simulink model "sys1"  (R2023b)
settings: Solver=VariableStepAuto  StartTime=0.0  StopTime=30e-3  RelTol=1e-3
InitFcn:
  | fs = 100e6;
  | ts = 1 / fs;
values from neighbouring files (symbols this model uses):
  c = 3e8    (= 300000000)    [init_param.m]
  H_az1 = zeros(numSamples,numPulses)    [init_param.m]
  H_az2 = zeros(numSamples,numPulses)    [init_param.m]
  H_ref = fft(conj(fliplr(txChirp)), numSamples)    [init_param.m]
  rawData = rawData + 0.01 * (randn(size(rawData)) + 1j * randn(size(rawData)))    [init_param.m]
  x1 = zeros(size(rawData))    [main.m]
  x2 = zeros(size(x1))    [main.m]
  x3 = zeros(size(x2))    [main.m]
  x4 = zeros(size(x3))    [main.m]
  x5 = zeros(size(x4))    [main.m]
  x6 = zeros(size(x5))    [main.m]
  xx4 = zeros(size(xx3))    [main.m]
  xx5 = zeros(size(xx4))    [main.m]
  xx6 = zeros(size(xx5))    [main.m]
undefined symbols (not defined in the file or in its folder): ffva1156, w2, w3, w4, w5, w6, w7, w8, w9, ww2, ww3, ww4, ww5, ww6, ww7, ww8, ww9, xcku095
libraries: hdlBasic x917, hdlDSPIP x18, dspsrcs4 x12, vmcUtilities x1
(part 6 of 9)

== system sys1/SAR/stream/stream_fft/stage8/BF ==
  re2 : Inport
  im2 : Inport  Port=2
  re1 : Inport  Port=3
  im1 : Inport  Port=4
  AddSub1 : hdlBasic/AddSub  mode=Addition  use_carryin=off  use_carryout=off  en=off  latency=0  precision=User Defined  arith_type="Signed  (2's comp)"  n_bits=16  bin_pt=0  quantization="Round  (unbiased: +/- Inf)"  overflow=Flag as error  use_behavioral_HDL=off  hw_selection=Fabric  pipelined=off  XmcBlockStatus=1  maskContainerNames=tabcontainer1  block_type=addsub  block_config=sysgen:Addsub_config
  AddSub2 : hdlBasic/AddSub  mode=Addition  use_carryin=off  use_carryout=off  en=off  latency=0  precision=User Defined  arith_type="Signed  (2's comp)"  n_bits=16  bin_pt=0  quantization="Round  (unbiased: +/- Inf)"  overflow=Flag as error  use_behavioral_HDL=off  hw_selection=Fabric  pipelined=off  XmcBlockStatus=1  maskContainerNames=tabcontainer1  block_type=addsub  block_config=sysgen:Addsub_config
  AddSub3 : hdlBasic/AddSub  mode=Subtraction  use_carryin=off  use_carryout=off  en=off  latency=0  precision=User Defined  arith_type="Signed  (2's comp)"  n_bits=16  bin_pt=0  quantization="Round  (unbiased: +/- Inf)"  overflow=Flag as error  use_behavioral_HDL=off  hw_selection=Fabric  pipelined=off  XmcBlockStatus=1  maskContainerNames=tabcontainer1  block_type=addsub  block_config=sysgen:Addsub_config
  AddSub4 : hdlBasic/AddSub  mode=Subtraction  use_carryin=off  use_carryout=off  en=off  latency=0  precision=User Defined  arith_type="Signed  (2's comp)"  n_bits=16  bin_pt=0  quantization="Round  (unbiased: +/- Inf)"  overflow=Flag as error  use_behavioral_HDL=off  hw_selection=Fabric  pipelined=off  XmcBlockStatus=1  maskContainerNames=tabcontainer1  block_type=addsub  block_config=sysgen:Addsub_config
  Delay2 : hdlBasic/Delay  rst=off  en=off  latency=7  reg_retiming=off  XmcBlockStatus=1  maskContainerNames=group1  block_type=delay  block_config=sysgen:Delay_config
  Delay3 : hdlBasic/Delay  rst=off  en=off  latency=7  reg_retiming=off  XmcBlockStatus=1  maskContainerNames=group1  block_type=delay  block_config=sysgen:Delay_config
  Out2_r : Outport
  Out2_i : Outport  Port=2
  Out1_r : Outport  Port=3
  Out1_i : Outport  Port=4
  wires:
  Delay3/1 -> Out2_i/1
  Delay2/1 -> Out2_r/1
  im1/1 -> AddSub3/2, AddSub1/2
  re1/1 -> AddSub4/2, AddSub2/2
  AddSub1/1 -> Delay3/1
  AddSub2/1 -> Delay2/1
  im2/1 -> AddSub3/1, AddSub1/1
  re2/1 -> AddSub4/1, AddSub2/1
  AddSub3/1 -> Out1_i/1
  AddSub4/1 -> Out1_r/1

== system sys1/SAR/stream/stream_fft/stage8/Multiplexer ==
  r1 : Inport
  i1 : Inport  Port=2
  r2 : Inport  Port=3
  i2 : Inport  Port=4
  cnt : Inport  Port=5
  BitBasher : hdlBasic/BitBasher  bitexpr=a={b[17]}  display_expr=off  sr_1=a  arith_type1=Unsigned  bin_pt1=0  sr_2=2  arith_type2=Unsigned  bin_pt2=0  sr_3=3  arith_type3=Unsigned  bin_pt3=0  sr_4=4  arith_type4=Unsigned  bin_pt4=0  XmcBlockStatus=1  maskContainerNames=group1  block_type=bitbasher  block_config=sysgen:BitBasher_config
  Inverter : hdlBasic/Inverter  en=off  latency=0  XmcBlockStatus=1  maskContainerNames=group2  block_type=inv  block_config=sysgen:Inverter_config
  Mux : hdlBasic/Mux  inputs=2  en=off  latency=0  precision=Full  arith_type=Unsigned  n_bits=16  bin_pt=14  quantization=Truncate  overflow=Wrap  XmcBlockStatus=1  maskContainerNames=tabcontainer1  block_type=mux  block_config=sysgen:Mux_config
  Mux1 : hdlBasic/Mux  inputs=2  en=off  latency=0  precision=Full  arith_type=Unsigned  n_bits=16  bin_pt=14  quantization=Truncate  overflow=Wrap  XmcBlockStatus=1  maskContainerNames=tabcontainer1  block_type=mux  block_config=sysgen:Mux_config
  rr : Outport
  ii : Outport  Port=2
  wires:
  Inverter/1 -> Mux1/1, Mux/1
  cnt/1 -> BitBasher/1
  Mux/1 -> rr/1
  Mux1/1 -> ii/1
  i1/1 -> Mux1/3
  r2/1 -> Mux/2
  BitBasher/1 -> Inverter/1
  i2/1 -> Mux1/2
  r1/1 -> Mux/3

== system sys1/SAR/stream/stream_fft/stage8/Twiddle ==
  r : Inport
  i : Inport  Port=2
  cnt : Inport  Port=3
  BitBasher1 : hdlBasic/BitBasher  bitexpr=a={b[16:10]}  display_expr=off  sr_1=a  arith_type1=Unsigned  bin_pt1=0  sr_2=2  arith_type2=Unsigned  bin_pt2=0  sr_3=3  arith_type3=Unsigned  bin_pt3=0  sr_4=4  arith_type4=Unsigned  bin_pt4=0  XmcBlockStatus=1  maskContainerNames=group1  block_type=bitbasher  block_config=sysgen:BitBasher_config
  Complex Multiplier 6.0 : hdlDSPIP/Complex Multiplier 6.0   hasatlast=off  hasatuser=off  atuserwidth=1  hasbtlast=off  hasbtuser=off  btuserwidth=1  multtype=Use_Mults  optimizegoal=Resources  flowcontrol=NonBlocking  outputwidth=32  roundmode=Truncate  hasctrltlast=off  hasctrltuser=off  ctrltuserwidth=1  outtlastbehv=Null  latencyconfig=Manual  minimumlatency=6  aclken=off  aresetn=off  trim_axipin_name=on  simulation_type=hybrid_sim  simulation_model=sysgen:cmpy_v6_0  data_path_portlist={ 's_axis_a_tdata_real', 's_axis_a_tdata_imag', 's_axis_b_tdata_real', 's_axis_b_tdata_imag', 's_axis_ctrl_tdata_rounding_bit', 'm_axis_dout_tdata_real', 'm_axis_dout_tdata_imag' }  aportwidth=63  bportwidth=63  ip_name=Complex Multiplier  ip_version=6.0  dsptool_ready=true  ipcore_usecache=true  ipcore_useipmodelcache=true  ipcore_verbose=false  ipcore_latency_parameter='minimumlatency'  wrapper_available=true  port_translation_map={ 'aclken' => 'en', 'aresetn' => 'rst'}  XmcBlockStatus=1  maskContainerNames=tabcontainer1  block_type=cmpy_v6_0  block_config=sysgen:rodinimport_config
  Constant2 : hdlBasic/Constant  const=1  gui_display_data_type=Boolean  arith_type=Boolean  n_bits=16  bin_pt=14  preci_type=Single  exp_width=8  frac_width=24  explicit_period=on  period=ts  XmcBlockStatus=1  maskContainerNames=tabcontainer1  block_type=constant  block_config=sysgen:Constant_config
  Constant3 : hdlBasic/Constant  const=1  gui_display_data_type=Boolean  arith_type=Boolean  n_bits=16  bin_pt=14  preci_type=Single  exp_width=8  frac_width=24  explicit_period=on  period=ts  XmcBlockStatus=1  maskContainerNames=tabcontainer1  block_type=constant  block_config=sysgen:Constant_config
  Convert1 : hdlBasic/Convert  gui_display_data_type=Fixed-point  arith_type=Signed (2's comp)  n_bits=16  bin_pt=0  float_type=Single  exp_bits=8  fraction_bits=24  quantization=Truncate  overflow=Flag as error  en=off  latency=0  pipeline=off  XmcBlockStatus=1  maskContainerNames=group2  block_type=convert  block_config=sysgen:Convert_config  block_width=595  block_height=885
  Convert2 : hdlBasic/Convert  gui_display_data_type=Fixed-point  arith_type=Signed (2's comp)  n_bits=16  bin_pt=0  float_type=Single  exp_bits=8  fraction_bits=24  quantization=Truncate  overflow=Flag as error  en=off  latency=0  pipeline=off  XmcBlockStatus=1  maskContainerNames=group2  block_type=convert  block_config=sysgen:Convert_config  block_width=595  block_height=885
  Delay2 : hdlBasic/Delay  rst=off  en=off  latency=1  reg_retiming=off  XmcBlockStatus=1  maskContainerNames=group1  block_type=delay  block_config=sysgen:Delay_config
  Delay3 : hdlBasic/Delay  rst=off  en=off  latency=1  reg_retiming=off  XmcBlockStatus=1  maskContainerNames=group1  block_type=delay  block_config=sysgen:Delay_config
  ROM : hdlBasic/ROM  depth=length(w8)  initVector=real(w8)  distributed_mem=Block RAM  rst=off  init_reg=0  en=off  latency=1  gui_display_data_type=Fixed-point  arith_type="Signed  (2's comp)"  n_bits=16  bin_pt=15  preci_type=Single  exp_width=8  frac_width=24  optimize=Area  use_rpm=on  simulation_type=fast_sim  XmcBlockStatus=1  maskContainerNames=tabcontainer1  block_type=sprom  block_config=sysgen:SPROM_config
  ROM1 : hdlBasic/ROM  depth=length(w8)  initVector=imag(w8)  distributed_mem=Block RAM  rst=off  init_reg=0  en=off  latency=1  gui_display_data_type=Fixed-point  arith_type="Signed  (2's comp)"  n_bits=16  bin_pt=15  preci_type=Single  exp_width=8  frac_width=24  optimize=Area  use_rpm=on  simulation_type=fast_sim  XmcBlockStatus=1  maskContainerNames=tabcontainer1  block_type=sprom  block_config=sysgen:SPROM_config
  rr : Outport
  ii : Outport  Port=2
  wires:
  Delay3/1 -> Complex Multiplier 6.0/3
  Delay2/1 -> Complex Multiplier 6.0/2
  Convert1/1 -> rr/1
  Convert2/1 -> ii/1
  cnt/1 -> BitBasher1/1
  r/1 -> Delay3/1
  Complex Multiplier 6.0/3 -> Convert1/1
  i/1 -> Delay2/1
  Constant3/1 -> Complex Multiplier 6.0/4
  ROM/1 -> Complex Multiplier 6.0/6
  Constant2/1 -> Complex Multiplier 6.0/1
  Complex Multiplier 6.0/2 -> Convert2/1
  BitBasher1/1 -> ROM1/1, ROM/1
  ROM1/1 -> Complex Multiplier 6.0/5

== system sys1/SAR/stream/stream_fft/stage8/delay ==
  r : Inport
  i : Inport  Port=2
  cnt : Inport  Port=3
  r1 : Inport  Port=4
  i1 : Inport  Port=5
  BitBasher : hdlBasic/BitBasher  bitexpr=a={b[17]}  display_expr=off  sr_1=a  arith_type1=Unsigned  bin_pt1=0  sr_2=2  arith_type2=Unsigned  bin_pt2=0  sr_3=3  arith_type3=Unsigned  bin_pt3=0  sr_4=4  arith_type4=Unsigned  bin_pt4=0  XmcBlockStatus=1  maskContainerNames=group1  block_type=bitbasher  block_config=sysgen:BitBasher_config
  Inverter : hdlBasic/Inverter  en=off  latency=0  XmcBlockStatus=1  maskContainerNames=group2  block_type=inv  block_config=sysgen:Inverter_config
  Mux : hdlBasic/Mux  inputs=2  en=off  latency=0  precision=Full  arith_type=Unsigned  n_bits=16  bin_pt=14  quantization=Truncate  overflow=Wrap  XmcBlockStatus=1  maskContainerNames=tabcontainer1  block_type=mux  block_config=sysgen:Mux_config
  Mux1 : hdlBasic/Mux  inputs=2  en=off  latency=0  precision=Full  arith_type=Unsigned  n_bits=16  bin_pt=14  quantization=Truncate  overflow=Wrap  XmcBlockStatus=1  maskContainerNames=tabcontainer1  block_type=mux  block_config=sysgen:Mux_config
  delay : Subsystem
  delay1 : Subsystem
  rr : Outport
  ii : Outport  Port=2
  wires:
  i/1 -> Mux1/3
  r/1 -> Mux/3
  delay1/1(out) -> ii/1
  delay/1(out) -> rr/1
  i1/1 -> Mux1/2
  r1/1 -> Mux/2
  Mux1/1 -> delay1/1(in)
  Mux/1 -> delay/1(in)
  BitBasher/1 -> Inverter/1
  cnt/1 -> BitBasher/1
  Inverter/1 -> Mux/1, Mux1/1

== system sys1/SAR/stream/stream_fft/stage9/BF ==
  re2 : Inport
  im2 : Inport  Port=2
  re1 : Inport  Port=3
  im1 : Inport  Port=4
  AddSub1 : hdlBasic/AddSub  mode=Addition  use_carryin=off  use_carryout=off  en=off  latency=0  precision=User Defined  arith_type="Signed  (2's comp)"  n_bits=16  bin_pt=0  quantization="Round  (unbiased: +/- Inf)"  overflow=Flag as error  use_behavioral_HDL=off  hw_selection=Fabric  pipelined=off  XmcBlockStatus=1  maskContainerNames=tabcontainer1  block_type=addsub  block_config=sysgen:Addsub_config
  AddSub2 : hdlBasic/AddSub  mode=Addition  use_carryin=off  use_carryout=off  en=off  latency=0  precision=User Defined  arith_type="Signed  (2's comp)"  n_bits=16  bin_pt=0  quantization="Round  (unbiased: +/- Inf)"  overflow=Flag as error  use_behavioral_HDL=off  hw_selection=Fabric  pipelined=off  XmcBlockStatus=1  maskContainerNames=tabcontainer1  block_type=addsub  block_config=sysgen:Addsub_config
  AddSub3 : hdlBasic/AddSub  mode=Subtraction  use_carryin=off  use_carryout=off  en=off  latency=0  precision=User Defined  arith_type="Signed  (2's comp)"  n_bits=16  bin_pt=0  quantization="Round  (unbiased: +/- Inf)"  overflow=Flag as error  use_behavioral_HDL=off  hw_selection=Fabric  pipelined=off  XmcBlockStatus=1  maskContainerNames=tabcontainer1  block_type=addsub  block_config=sysgen:Addsub_config
  AddSub4 : hdlBasic/AddSub  mode=Subtraction  use_carryin=off  use_carryout=off  en=off  latency=0  precision=User Defined  arith_type="Signed  (2's comp)"  n_bits=16  bin_pt=0  quantization="Round  (unbiased: +/- Inf)"  overflow=Flag as error  use_behavioral_HDL=off  hw_selection=Fabric  pipelined=off  XmcBlockStatus=1  maskContainerNames=tabcontainer1  block_type=addsub  block_config=sysgen:Addsub_config
  Delay2 : hdlBasic/Delay  rst=off  en=off  latency=7  reg_retiming=off  XmcBlockStatus=1  maskContainerNames=group1  block_type=delay  block_config=sysgen:Delay_config
  Delay3 : hdlBasic/Delay  rst=off  en=off  latency=7  reg_retiming=off  XmcBlockStatus=1  maskContainerNames=group1  block_type=delay  block_config=sysgen:Delay_config
  Out2_r : Outport
  Out2_i : Outport  Port=2
  Out1_r : Outport  Port=3
  Out1_i : Outport  Port=4
  wires:
  AddSub4/1 -> Out1_r/1
  AddSub3/1 -> Out1_i/1
  re2/1 -> AddSub2/1, AddSub4/1
  im2/1 -> AddSub1/1, AddSub3/1
  AddSub2/1 -> Delay2/1
  AddSub1/1 -> Delay3/1
  re1/1 -> AddSub2/2, AddSub4/2
  im1/1 -> AddSub1/2, AddSub3/2
  Delay2/1 -> Out2_r/1
  Delay3/1 -> Out2_i/1

== system sys1/SAR/stream/stream_fft/stage9/Multiplexer ==
  r1 : Inport
  i1 : Inport  Port=2
  r2 : Inport  Port=3
  i2 : Inport  Port=4
  cnt : Inport  Port=5
  BitBasher : hdlBasic/BitBasher  bitexpr=a={b[18]}  display_expr=off  sr_1=a  arith_type1=Unsigned  bin_pt1=0  sr_2=2  arith_type2=Unsigned  bin_pt2=0  sr_3=3  arith_type3=Unsigned  bin_pt3=0  sr_4=4  arith_type4=Unsigned  bin_pt4=0  XmcBlockStatus=1  maskContainerNames=group1  block_type=bitbasher  block_config=sysgen:BitBasher_config
  Inverter : hdlBasic/Inverter  en=off  latency=0  XmcBlockStatus=1  maskContainerNames=group2  block_type=inv  block_config=sysgen:Inverter_config
  Mux : hdlBasic/Mux  inputs=2  en=off  latency=0  precision=Full  arith_type=Unsigned  n_bits=16  bin_pt=14  quantization=Truncate  overflow=Wrap  XmcBlockStatus=1  maskContainerNames=tabcontainer1  block_type=mux  block_config=sysgen:Mux_config
  Mux1 : hdlBasic/Mux  inputs=2  en=off  latency=0  precision=Full  arith_type=Unsigned  n_bits=16  bin_pt=14  quantization=Truncate  overflow=Wrap  XmcBlockStatus=1  maskContainerNames=tabcontainer1  block_type=mux  block_config=sysgen:Mux_config
  rr : Outport
  ii : Outport  Port=2
  wires:
  r1/1 -> Mux/3
  i2/1 -> Mux1/2
  BitBasher/1 -> Inverter/1
  r2/1 -> Mux/2
  i1/1 -> Mux1/3
  Mux1/1 -> ii/1
  Mux/1 -> rr/1
  cnt/1 -> BitBasher/1
  Inverter/1 -> Mux/1, Mux1/1

== system sys1/SAR/stream/stream_fft/stage9/Twiddle ==
  r : Inport
  i : Inport  Port=2
  cnt : Inport  Port=3
  BitBasher1 : hdlBasic/BitBasher  bitexpr=a={b[17:10]}  display_expr=off  sr_1=a  arith_type1=Unsigned  bin_pt1=0  sr_2=2  arith_type2=Unsigned  bin_pt2=0  sr_3=3  arith_type3=Unsigned  bin_pt3=0  sr_4=4  arith_type4=Unsigned  bin_pt4=0  XmcBlockStatus=1  maskContainerNames=group1  block_type=bitbasher  block_config=sysgen:BitBasher_config
  Complex Multiplier 6.0 : hdlDSPIP/Complex Multiplier 6.0   hasatlast=off  hasatuser=off  atuserwidth=1  hasbtlast=off  hasbtuser=off  btuserwidth=1  multtype=Use_Mults  optimizegoal=Resources  flowcontrol=NonBlocking  outputwidth=32  roundmode=Truncate  hasctrltlast=off  hasctrltuser=off  ctrltuserwidth=1  outtlastbehv=Null  latencyconfig=Manual  minimumlatency=6  aclken=off  aresetn=off  trim_axipin_name=on  simulation_type=hybrid_sim  simulation_model=sysgen:cmpy_v6_0  data_path_portlist={ 's_axis_a_tdata_real', 's_axis_a_tdata_imag', 's_axis_b_tdata_real', 's_axis_b_tdata_imag', 's_axis_ctrl_tdata_rounding_bit', 'm_axis_dout_tdata_real', 'm_axis_dout_tdata_imag' }  aportwidth=63  bportwidth=63  ip_name=Complex Multiplier  ip_version=6.0  dsptool_ready=true  ipcore_usecache=true  ipcore_useipmodelcache=true  ipcore_verbose=false  ipcore_latency_parameter='minimumlatency'  wrapper_available=true  port_translation_map={ 'aclken' => 'en', 'aresetn' => 'rst'}  XmcBlockStatus=1  maskContainerNames=tabcontainer1  block_type=cmpy_v6_0  block_config=sysgen:rodinimport_config
  Constant2 : hdlBasic/Constant  const=1  gui_display_data_type=Boolean  arith_type=Boolean  n_bits=16  bin_pt=14  preci_type=Single  exp_width=8  frac_width=24  explicit_period=on  period=ts  XmcBlockStatus=1  maskContainerNames=tabcontainer1  block_type=constant  block_config=sysgen:Constant_config
  Constant3 : hdlBasic/Constant  const=1  gui_display_data_type=Boolean  arith_type=Boolean  n_bits=16  bin_pt=14  preci_type=Single  exp_width=8  frac_width=24  explicit_period=on  period=ts  XmcBlockStatus=1  maskContainerNames=tabcontainer1  block_type=constant  block_config=sysgen:Constant_config
  Convert1 : hdlBasic/Convert  gui_display_data_type=Fixed-point  arith_type=Signed (2's comp)  n_bits=16  bin_pt=0  float_type=Single  exp_bits=8  fraction_bits=24  quantization=Truncate  overflow=Flag as error  en=off  latency=0  pipeline=off  XmcBlockStatus=1  maskContainerNames=group2  block_type=convert  block_config=sysgen:Convert_config  block_width=595  block_height=885
  Convert2 : hdlBasic/Convert  gui_display_data_type=Fixed-point  arith_type=Signed (2's comp)  n_bits=16  bin_pt=0  float_type=Single  exp_bits=8  fraction_bits=24  quantization=Truncate  overflow=Flag as error  en=off  latency=0  pipeline=off  XmcBlockStatus=1  maskContainerNames=group2  block_type=convert  block_config=sysgen:Convert_config  block_width=595  block_height=885
  Delay2 : hdlBasic/Delay  rst=off  en=off  latency=1  reg_retiming=off  XmcBlockStatus=1  maskContainerNames=group1  block_type=delay  block_config=sysgen:Delay_config
  Delay3 : hdlBasic/Delay  rst=off  en=off  latency=1  reg_retiming=off  XmcBlockStatus=1  maskContainerNames=group1  block_type=delay  block_config=sysgen:Delay_config
  ROM : hdlBasic/ROM  depth=length(w9)  initVector=real(w9)  distributed_mem=Block RAM  rst=off  init_reg=0  en=off  latency=1  gui_display_data_type=Fixed-point  arith_type="Signed  (2's comp)"  n_bits=16  bin_pt=15  preci_type=Single  exp_width=8  frac_width=24  optimize=Area  use_rpm=on  simulation_type=fast_sim  XmcBlockStatus=1  maskContainerNames=tabcontainer1  block_type=sprom  block_config=sysgen:SPROM_config
  ROM1 : hdlBasic/ROM  depth=length(w9)  initVector=imag(w9)  distributed_mem=Block RAM  rst=off  init_reg=0  en=off  latency=1  gui_display_data_type=Fixed-point  arith_type="Signed  (2's comp)"  n_bits=16  bin_pt=15  preci_type=Single  exp_width=8  frac_width=24  optimize=Area  use_rpm=on  simulation_type=fast_sim  XmcBlockStatus=1  maskContainerNames=tabcontainer1  block_type=sprom  block_config=sysgen:SPROM_config
  rr : Outport
  ii : Outport  Port=2
  wires:
  ROM1/1 -> Complex Multiplier 6.0/5
  BitBasher1/1 -> ROM/1, ROM1/1
  Complex Multiplier 6.0/2 -> Convert2/1
  Constant2/1 -> Complex Multiplier 6.0/1
  ROM/1 -> Complex Multiplier 6.0/6
  Constant3/1 -> Complex Multiplier 6.0/4
  i/1 -> Delay2/1
  Complex Multiplier 6.0/3 -> Convert1/1
  r/1 -> Delay3/1
  cnt/1 -> BitBasher1/1
  Convert2/1 -> ii/1
  Convert1/1 -> rr/1
  Delay2/1 -> Complex Multiplier 6.0/2
  Delay3/1 -> Complex Multiplier 6.0/3

== system sys1/SAR/stream/stream_fft/stage9/delay ==
  r : Inport
  i : Inport  Port=2
  cnt : Inport  Port=3
  r1 : Inport  Port=4
  i1 : Inport  Port=5
  BitBasher : hdlBasic/BitBasher  bitexpr=a={b[18]}  display_expr=off  sr_1=a  arith_type1=Unsigned  bin_pt1=0  sr_2=2  arith_type2=Unsigned  bin_pt2=0  sr_3=3  arith_type3=Unsigned  bin_pt3=0  sr_4=4  arith_type4=Unsigned  bin_pt4=0  XmcBlockStatus=1  maskContainerNames=group1  block_type=bitbasher  block_config=sysgen:BitBasher_config
  Inverter : hdlBasic/Inverter  en=off  latency=0  XmcBlockStatus=1  maskContainerNames=group2  block_type=inv  block_config=sysgen:Inverter_config
  Mux : hdlBasic/Mux  inputs=2  en=off  latency=0  precision=Full  arith_type=Unsigned  n_bits=16  bin_pt=14  quantization=Truncate  overflow=Wrap  XmcBlockStatus=1  maskContainerNames=tabcontainer1  block_type=mux  block_config=sysgen:Mux_config
  Mux1 : hdlBasic/Mux  inputs=2  en=off  latency=0  precision=Full  arith_type=Unsigned  n_bits=16  bin_pt=14  quantization=Truncate  overflow=Wrap  XmcBlockStatus=1  maskContainerNames=tabcontainer1  block_type=mux  block_config=sysgen:Mux_config
  delay : Subsystem
  delay1 : Subsystem
  rr : Outport
  ii : Outport  Port=2
  wires:
  Inverter/1 -> Mux1/1, Mux/1
  cnt/1 -> BitBasher/1
  BitBasher/1 -> Inverter/1
  Mux/1 -> delay/1(in)
  Mux1/1 -> delay1/1(in)
  r1/1 -> Mux/2
  i1/1 -> Mux1/2
  delay/1(out) -> rr/1
  delay1/1(out) -> ii/1
  r/1 -> Mux/3
  i/1 -> Mux1/3

== system sys1/SAR/stream/stream_ifft/stage1/BF ==
  ur : Inport
  ui : Inport  Port=2
  vr : Inport  Port=3
  vi : Inport  Port=4
  AddSub1 : hdlBasic/AddSub  mode=Addition  use_carryin=off  use_carryout=off  en=off  latency=0  precision=User Defined  arith_type="Signed  (2's comp)"  n_bits=16  bin_pt=0  quantization="Round  (unbiased: +/- Inf)"  overflow=Flag as error  use_behavioral_HDL=off  hw_selection=Fabric  pipelined=off  XmcBlockStatus=1  maskContainerNames=tabcontainer1  block_type=addsub  block_config=sysgen:Addsub_config
  AddSub2 : hdlBasic/AddSub  mode=Addition  use_carryin=off  use_carryout=off  en=off  latency=0  precision=User Defined  arith_type="Signed  (2's comp)"  n_bits=16  bin_pt=0  quantization="Round  (unbiased: +/- Inf)"  overflow=Flag as error  use_behavioral_HDL=off  hw_selection=Fabric  pipelined=off  XmcBlockStatus=1  maskContainerNames=tabcontainer1  block_type=addsub  block_config=sysgen:Addsub_config
  AddSub3 : hdlBasic/AddSub  mode=Subtraction  use_carryin=off  use_carryout=off  en=off  latency=0  precision=User Defined  arith_type="Signed  (2's comp)"  n_bits=16  bin_pt=0  quantization="Round  (unbiased: +/- Inf)"  overflow=Flag as error  use_behavioral_HDL=off  hw_selection=Fabric  pipelined=off  XmcBlockStatus=1  maskContainerNames=tabcontainer1  block_type=addsub  block_config=sysgen:Addsub_config
  AddSub4 : hdlBasic/AddSub  mode=Subtraction  use_carryin=off  use_carryout=off  en=off  latency=0  precision=User Defined  arith_type="Signed  (2's comp)"  n_bits=16  bin_pt=0  quantization="Round  (unbiased: +/- Inf)"  overflow=Flag as error  use_behavioral_HDL=off  hw_selection=Fabric  pipelined=off  XmcBlockStatus=1  maskContainerNames=tabcontainer1  block_type=addsub  block_config=sysgen:Addsub_config
  Out2_r : Outport
  Out2_i : Outport  Port=2
  Out1_r : Outport  Port=3
  Out1_i : Outport  Port=4
  wires:
  AddSub2/1 -> Out2_r/1
  AddSub1/1 -> Out2_i/1
  AddSub3/1 -> Out1_r/1
  AddSub4/1 -> Out1_i/1
  ur/1 -> AddSub2/1, AddSub3/1
  ui/1 -> AddSub1/1, AddSub4/1
  vr/1 -> AddSub2/2, AddSub3/2
  vi/1 -> AddSub1/2, AddSub4/2

== system sys1/SAR/stream/stream_ifft/stage1/Multiplexer ==
  r2 : Inport
  i2 : Inport  Port=2
  r1 : Inport  Port=3
  i1 : Inport  Port=4
  cnt : Inport  Port=5
  BitBasher : hdlBasic/BitBasher  bitexpr=a={b[10]}  display_expr=on  sr_1=a  arith_type1=Unsigned  bin_pt1=0  sr_2=2  arith_type2=Unsigned  bin_pt2=0  sr_3=3  arith_type3=Unsigned  bin_pt3=0  sr_4=4  arith_type4=Unsigned  bin_pt4=0  XmcBlockStatus=1  maskContainerNames=group1  block_type=bitbasher  block_config=sysgen:BitBasher_config
  Delay1 : hdlBasic/Delay  rst=off  en=off  latency=7  reg_retiming=off  XmcBlockStatus=1  maskContainerNames=group1  block_type=delay  block_config=sysgen:Delay_config
  Inverter : hdlBasic/Inverter  en=off  latency=0  XmcBlockStatus=1  maskContainerNames=group2  block_type=inv  block_config=sysgen:Inverter_config
  Mux : hdlBasic/Mux  inputs=2  en=off  latency=0  precision=Full  arith_type=Unsigned  n_bits=16  bin_pt=14  quantization=Truncate  overflow=Wrap  XmcBlockStatus=1  maskContainerNames=tabcontainer1  block_type=mux  block_config=sysgen:Mux_config
  Mux1 : hdlBasic/Mux  inputs=2  en=off  latency=0  precision=Full  arith_type=Unsigned  n_bits=16  bin_pt=14  quantization=Truncate  overflow=Wrap  XmcBlockStatus=1  maskContainerNames=tabcontainer1  block_type=mux  block_config=sysgen:Mux_config
  rr : Outport
  ii : Outport  Port=2
  wires:
  Delay1/1 -> Mux1/1, Mux/1
  Inverter/1 -> Delay1/1
  r1/1 -> Mux/2
  r2/1 -> Mux/3
  i2/1 -> Mux1/3
  i1/1 -> Mux1/2
  cnt/1 -> BitBasher/1
  Mux/1 -> rr/1
  Mux1/1 -> ii/1
  BitBasher/1 -> Inverter/1

== system sys1/SAR/stream/stream_ifft/stage1/Twiddle1 ==
  r : Inport
  i : Inport  Port=2
  cnt : Inport  Port=3
  Delay1 : hdlBasic/Delay  rst=off  en=off  latency=6  reg_retiming=off  XmcBlockStatus=1  maskContainerNames=group1  block_type=delay  block_config=sysgen:Delay_config
  Delay7 : hdlBasic/Delay  rst=off  en=off  latency=6  reg_retiming=off  XmcBlockStatus=1  maskContainerNames=group1  block_type=delay  block_config=sysgen:Delay_config
  rr : Outport
  ii : Outport  Port=2
  wires:
  r/1 -> Delay1/1
  i/1 -> Delay7/1
  Delay7/1 -> ii/1
  Delay1/1 -> rr/1

== system sys1/SAR/stream/stream_ifft/stage1/delay ==
  r : Inport
  i : Inport  Port=2
  cnt : Inport  Port=3
  r1 : Inport  Port=4
  i1 : Inport  Port=5
  BitBasher : hdlBasic/BitBasher  bitexpr=a={b[10]}  display_expr=off  sr_1=a  arith_type1=Unsigned  bin_pt1=0  sr_2=2  arith_type2=Unsigned  bin_pt2=0  sr_3=3  arith_type3=Unsigned  bin_pt3=0  sr_4=4  arith_type4=Unsigned  bin_pt4=0  XmcBlockStatus=1  maskContainerNames=group1  block_type=bitbasher  block_config=sysgen:BitBasher_config
  Delay4 : hdlBasic/Delay  rst=off  en=off  latency=6  reg_retiming=off  XmcBlockStatus=1  maskContainerNames=group1  block_type=delay  block_config=sysgen:Delay_config
  Delay6 : hdlBasic/Delay  rst=off  en=off  latency=6  reg_retiming=off  XmcBlockStatus=1  maskContainerNames=group1  block_type=delay  block_config=sysgen:Delay_config
  Delay9 : hdlBasic/Delay  rst=off  en=off  latency=7  reg_retiming=off  XmcBlockStatus=1  maskContainerNames=group1  block_type=delay  block_config=sysgen:Delay_config
  Inverter : hdlBasic/Inverter  en=off  latency=0  XmcBlockStatus=1  maskContainerNames=group2  block_type=inv  block_config=sysgen:Inverter_config
  Mux : hdlBasic/Mux  inputs=2  en=off  latency=0  precision=Full  arith_type=Unsigned  n_bits=16  bin_pt=14  quantization=Truncate  overflow=Wrap  XmcBlockStatus=1  maskContainerNames=tabcontainer1  block_type=mux  block_config=sysgen:Mux_config
  Mux1 : hdlBasic/Mux  inputs=2  en=off  latency=0  precision=Full  arith_type=Unsigned  n_bits=16  bin_pt=14  quantization=Truncate  overflow=Wrap  XmcBlockStatus=1  maskContainerNames=tabcontainer1  block_type=mux  block_config=sysgen:Mux_config
  delay : Subsystem
  delay1 : Subsystem
  rr : Outport
  ii : Outport  Port=2
  wires:
  Delay6/1 -> Mux1/3
  Delay4/1 -> Mux/3
  Delay9/1 -> Mux1/1, Mux/1
  r1/1 -> Mux/2
  i/1 -> Delay6/1
  Mux1/1 -> delay1/1(in)
  BitBasher/1 -> Inverter/1
  i1/1 -> Mux1/2
  r/1 -> Delay4/1
  delay/1(out) -> rr/1
  delay1/1(out) -> ii/1
  Mux/1 -> delay/1(in)
  cnt/1 -> BitBasher/1
  Inverter/1 -> Delay9/1

== system sys1/SAR/stream/stream_ifft/stage2/BF ==
  ur : Inport
  ui : Inport  Port=2
  vr : Inport  Port=3
  vi : Inport  Port=4
  AddSub1 : hdlBasic/AddSub  mode=Addition  use_carryin=off  use_carryout=off  en=off  latency=0  precision=User Defined  arith_type="Signed  (2's comp)"  n_bits=16  bin_pt=0  quantization="Round  (unbiased: +/- Inf)"  overflow=Flag as error  use_behavioral_HDL=off  hw_selection=Fabric  pipelined=off  XmcBlockStatus=1  maskContainerNames=tabcontainer1  block_type=addsub  block_config=sysgen:Addsub_config
  AddSub2 : hdlBasic/AddSub  mode=Addition  use_carryin=off  use_carryout=off  en=off  latency=0  precision=User Defined  arith_type="Signed  (2's comp)"  n_bits=16  bin_pt=0  quantization="Round  (unbiased: +/- Inf)"  overflow=Flag as error  use_behavioral_HDL=off  hw_selection=Fabric  pipelined=off  XmcBlockStatus=1  maskContainerNames=tabcontainer1  block_type=addsub  block_config=sysgen:Addsub_config
  AddSub3 : hdlBasic/AddSub  mode=Subtraction  use_carryin=off  use_carryout=off  en=off  latency=0  precision=User Defined  arith_type="Signed  (2's comp)"  n_bits=16  bin_pt=0  quantization="Round  (unbiased: +/- Inf)"  overflow=Flag as error  use_behavioral_HDL=off  hw_selection=Fabric  pipelined=off  XmcBlockStatus=1  maskContainerNames=tabcontainer1  block_type=addsub  block_config=sysgen:Addsub_config
  AddSub4 : hdlBasic/AddSub  mode=Subtraction  use_carryin=off  use_carryout=off  en=off  latency=0  precision=User Defined  arith_type="Signed  (2's comp)"  n_bits=16  bin_pt=0  quantization="Round  (unbiased: +/- Inf)"  overflow=Flag as error  use_behavioral_HDL=off  hw_selection=Fabric  pipelined=off  XmcBlockStatus=1  maskContainerNames=tabcontainer1  block_type=addsub  block_config=sysgen:Addsub_config
  Out2_r : Outport
  Out2_i : Outport  Port=2
  Out1_r : Outport  Port=3
  Out1_i : Outport  Port=4
  wires:
  AddSub2/1 -> Out2_r/1
  AddSub1/1 -> Out2_i/1
  AddSub3/1 -> Out1_r/1
  AddSub4/1 -> Out1_i/1
  ur/1 -> AddSub2/1, AddSub3/1
  ui/1 -> AddSub1/1, AddSub4/1
  vr/1 -> AddSub2/2, AddSub3/2
  vi/1 -> AddSub1/2, AddSub4/2

== system sys1/SAR/stream/stream_ifft/stage2/Multiplexer ==
  r2 : Inport
  i2 : Inport  Port=2
  r1 : Inport  Port=3
  i1 : Inport  Port=4
  cnt : Inport  Port=5
  BitBasher : hdlBasic/BitBasher  bitexpr=a={b[11]}  display_expr=on  sr_1=a  arith_type1=Unsigned  bin_pt1=0  sr_2=2  arith_type2=Unsigned  bin_pt2=0  sr_3=3  arith_type3=Unsigned  bin_pt3=0  sr_4=4  arith_type4=Unsigned  bin_pt4=0  XmcBlockStatus=1  maskContainerNames=group1  block_type=bitbasher  block_config=sysgen:BitBasher_config
  Delay1 : hdlBasic/Delay  rst=off  en=off  latency=7  reg_retiming=off  XmcBlockStatus=1  maskContainerNames=group1  block_type=delay  block_config=sysgen:Delay_config
  Inverter : hdlBasic/Inverter  en=off  latency=0  XmcBlockStatus=1  maskContainerNames=group2  block_type=inv  block_config=sysgen:Inverter_config
  Mux : hdlBasic/Mux  inputs=2  en=off  latency=0  precision=Full  arith_type=Unsigned  n_bits=16  bin_pt=14  quantization=Truncate  overflow=Wrap  XmcBlockStatus=1  maskContainerNames=tabcontainer1  block_type=mux  block_config=sysgen:Mux_config
  Mux1 : hdlBasic/Mux  inputs=2  en=off  latency=0  precision=Full  arith_type=Unsigned  n_bits=16  bin_pt=14  quantization=Truncate  overflow=Wrap  XmcBlockStatus=1  maskContainerNames=tabcontainer1  block_type=mux  block_config=sysgen:Mux_config
  rr : Outport
  ii : Outport  Port=2
  wires:
  BitBasher/1 -> Inverter/1
  Mux1/1 -> ii/1
  Mux/1 -> rr/1
  cnt/1 -> BitBasher/1
  i1/1 -> Mux1/2
  i2/1 -> Mux1/3
  r2/1 -> Mux/3
  r1/1 -> Mux/2
  Inverter/1 -> Delay1/1
  Delay1/1 -> Mux/1, Mux1/1

== system sys1/SAR/stream/stream_ifft/stage2/Twiddle1 ==
  r : Inport
  i : Inport  Port=2
  cnt : Inport  Port=3
  BitBasher1 : hdlBasic/BitBasher  bitexpr=a={b[10]}  display_expr=on  sr_1=a  arith_type1=Unsigned  bin_pt1=0  sr_2=2  arith_type2=Unsigned  bin_pt2=0  sr_3=3  arith_type3=Unsigned  bin_pt3=0  sr_4=4  arith_type4=Unsigned  bin_pt4=0  XmcBlockStatus=1  maskContainerNames=group1  block_type=bitbasher  block_config=sysgen:BitBasher_config
  Complex Multiplier 6.0 : hdlDSPIP/Complex Multiplier 6.0   hasatlast=off  hasatuser=off  atuserwidth=1  hasbtlast=off  hasbtuser=off  btuserwidth=1  multtype=Use_Mults  optimizegoal=Resources  flowcontrol=NonBlocking  outputwidth=33  roundmode=Truncate  hasctrltlast=off  hasctrltuser=off  ctrltuserwidth=1  outtlastbehv=Null  latencyconfig=Manual  minimumlatency=6  aclken=off  aresetn=off  trim_axipin_name=on  simulation_type=hybrid_sim  simulation_model=sysgen:cmpy_v6_0  data_path_portlist={ 's_axis_a_tdata_real', 's_axis_a_tdata_imag', 's_axis_b_tdata_real', 's_axis_b_tdata_imag', 's_axis_ctrl_tdata_rounding_bit', 'm_axis_dout_tdata_real', 'm_axis_dout_tdata_imag' }  aportwidth=63  bportwidth=63  ip_name=Complex Multiplier  ip_version=6.0  dsptool_ready=true  ipcore_usecache=true  ipcore_useipmodelcache=true  ipcore_verbose=false  ipcore_latency_parameter='minimumlatency'  wrapper_available=true  port_translation_map={ 'aclken' => 'en', 'aresetn' => 'rst'}  XmcBlockStatus=1  maskContainerNames=tabcontainer1  block_type=cmpy_v6_0  block_config=sysgen:rodinimport_config
  Constant2 : hdlBasic/Constant  const=1  gui_display_data_type=Boolean  arith_type=Boolean  n_bits=16  bin_pt=14  preci_type=Single  exp_width=8  frac_width=24  explicit_period=on  period=ts  XmcBlockStatus=1  maskContainerNames=tabcontainer1  block_type=constant  block_config=sysgen:Constant_config
  Constant3 : hdlBasic/Constant  const=1  gui_display_data_type=Boolean  arith_type=Boolean  n_bits=16  bin_pt=14  preci_type=Single  exp_width=8  frac_width=24  explicit_period=on  period=ts  XmcBlockStatus=1  maskContainerNames=tabcontainer1  block_type=constant  block_config=sysgen:Constant_config
  Convert : hdlBasic/Convert  gui_display_data_type=Fixed-point  arith_type=Signed (2's comp)  n_bits=16  bin_pt=0  float_type=Single  exp_bits=8  fraction_bits=24  quantization="Round  (unbiased: +/- Inf)"  overflow=Flag as error  en=off  latency=0  pipeline=off  XmcBlockStatus=1  maskContainerNames=group2  block_type=convert  block_config=sysgen:Convert_config  block_width=595  block_height=885
  Convert1 : hdlBasic/Convert  gui_display_data_type=Fixed-point  arith_type=Signed (2's comp)  n_bits=16  bin_pt=0  float_type=Single  exp_bits=8  fraction_bits=24  quantization="Round  (unbiased: +/- Inf)"  overflow=Flag as error  en=off  latency=0  pipeline=off  XmcBlockStatus=1  maskContainerNames=group2  block_type=convert  block_config=sysgen:Convert_config  block_width=595  block_height=885
  ROM : hdlBasic/ROM  depth=length(ww2)  initVector=real(ww2)  distributed_mem=Block RAM  rst=off  init_reg=0  en=off  latency=1  gui_display_data_type=Fixed-point  arith_type="Signed  (2's comp)"  n_bits=17  bin_pt=15  preci_type=Single  exp_width=8  frac_width=24  optimize=Area  use_rpm=on  simulation_type=fast_sim  XmcBlockStatus=1  maskContainerNames=tabcontainer1  block_type=sprom  block_config=sysgen:SPROM_config
  ROM1 : hdlBasic/ROM  depth=length(ww2)  initVector=imag(ww2)  distributed_mem=Block RAM  rst=off  init_reg=0  en=off  latency=1  gui_display_data_type=Fixed-point  arith_type="Signed  (2's comp)"  n_bits=17  bin_pt=15  preci_type=Single  exp_width=8  frac_width=24  optimize=Area  use_rpm=on  simulation_type=fast_sim  XmcBlockStatus=1  maskContainerNames=tabcontainer1  block_type=sprom  block_config=sysgen:SPROM_config
  rr : Outport
  ii : Outport  Port=2
  wires:
  Constant2/1 -> Complex Multiplier 6.0/1
  Constant3/1 -> Complex Multiplier 6.0/4
  BitBasher1/1 -> ROM/1, ROM1/1
  Complex Multiplier 6.0/3 -> Convert1/1
  Complex Multiplier 6.0/2 -> Convert/1
  Convert1/1 -> rr/1
  Convert/1 -> ii/1
  i/1 -> Complex Multiplier 6.0/2
  r/1 -> Complex Multiplier 6.0/3
  cnt/1 -> BitBasher1/1
  ROM1/1 -> Complex Multiplier 6.0/5
  ROM/1 -> Complex Multiplier 6.0/6

== system sys1/SAR/stream/stream_ifft/stage2/delay ==
  r : Inport
  i : Inport  Port=2
  cnt : Inport  Port=3
  r1 : Inport  Port=4
  i1 : Inport  Port=5
  BitBasher : hdlBasic/BitBasher  bitexpr=a={b[11]}  display_expr=off  sr_1=a  arith_type1=Unsigned  bin_pt1=0  sr_2=2  arith_type2=Unsigned  bin_pt2=0  sr_3=3  arith_type3=Unsigned  bin_pt3=0  sr_4=4  arith_type4=Unsigned  bin_pt4=0  XmcBlockStatus=1  maskContainerNames=group1  block_type=bitbasher  block_config=sysgen:BitBasher_config
  Delay4 : hdlBasic/Delay  rst=off  en=off  latency=6  reg_retiming=off  XmcBlockStatus=1  maskContainerNames=group1  block_type=delay  block_config=sysgen:Delay_config
  Delay6 : hdlBasic/Delay  rst=off  en=off  latency=6  reg_retiming=off  XmcBlockStatus=1  maskContainerNames=group1  block_type=delay  block_config=sysgen:Delay_config
  Delay9 : hdlBasic/Delay  rst=off  en=off  latency=7  reg_retiming=off  XmcBlockStatus=1  maskContainerNames=group1  block_type=delay  block_config=sysgen:Delay_config
  Inverter : hdlBasic/Inverter  en=off  latency=0  XmcBlockStatus=1  maskContainerNames=group2  block_type=inv  block_config=sysgen:Inverter_config
  Mux : hdlBasic/Mux  inputs=2  en=off  latency=0  precision=Full  arith_type=Unsigned  n_bits=16  bin_pt=14  quantization=Truncate  overflow=Wrap  XmcBlockStatus=1  maskContainerNames=tabcontainer1  block_type=mux  block_config=sysgen:Mux_config
  Mux1 : hdlBasic/Mux  inputs=2  en=off  latency=0  precision=Full  arith_type=Unsigned  n_bits=16  bin_pt=14  quantization=Truncate  overflow=Wrap  XmcBlockStatus=1  maskContainerNames=tabcontainer1  block_type=mux  block_config=sysgen:Mux_config
  delay : Subsystem
  delay1 : Subsystem
  rr : Outport
  ii : Outport  Port=2
  wires:
  Inverter/1 -> Delay9/1
  cnt/1 -> BitBasher/1
  Mux/1 -> delay/1(in)
  delay1/1(out) -> ii/1
  delay/1(out) -> rr/1
  r/1 -> Delay4/1
  i1/1 -> Mux1/2
  BitBasher/1 -> Inverter/1
  Mux1/1 -> delay1/1(in)
  i/1 -> Delay6/1
  r1/1 -> Mux/2
  Delay9/1 -> Mux/1, Mux1/1
  Delay4/1 -> Mux/3
  Delay6/1 -> Mux1/3

== system sys1/SAR/stream/stream_ifft/stage3/BF ==
  ur : Inport
  ui : Inport  Port=2
  vr : Inport  Port=3
  vi : Inport  Port=4
  AddSub1 : hdlBasic/AddSub  mode=Addition  use_carryin=off  use_carryout=off  en=off  latency=0  precision=User Defined  arith_type="Signed  (2's comp)"  n_bits=16  bin_pt=0  quantization="Round  (unbiased: +/- Inf)"  overflow=Flag as error  use_behavioral_HDL=off  hw_selection=Fabric  pipelined=off  XmcBlockStatus=1  maskContainerNames=tabcontainer1  block_type=addsub  block_config=sysgen:Addsub_config
  AddSub2 : hdlBasic/AddSub  mode=Addition  use_carryin=off  use_carryout=off  en=off  latency=0  precision=User Defined  arith_type="Signed  (2's comp)"  n_bits=16  bin_pt=0  quantization="Round  (unbiased: +/- Inf)"  overflow=Flag as error  use_behavioral_HDL=off  hw_selection=Fabric  pipelined=off  XmcBlockStatus=1  maskContainerNames=tabcontainer1  block_type=addsub  block_config=sysgen:Addsub_config
  AddSub3 : hdlBasic/AddSub  mode=Subtraction  use_carryin=off  use_carryout=off  en=off  latency=0  precision=User Defined  arith_type="Signed  (2's comp)"  n_bits=16  bin_pt=0  quantization="Round  (unbiased: +/- Inf)"  overflow=Flag as error  use_behavioral_HDL=off  hw_selection=Fabric  pipelined=off  XmcBlockStatus=1  maskContainerNames=tabcontainer1  block_type=addsub  block_config=sysgen:Addsub_config
  AddSub4 : hdlBasic/AddSub  mode=Subtraction  use_carryin=off  use_carryout=off  en=off  latency=0  precision=User Defined  arith_type="Signed  (2's comp)"  n_bits=16  bin_pt=0  quantization="Round  (unbiased: +/- Inf)"  overflow=Flag as error  use_behavioral_HDL=off  hw_selection=Fabric  pipelined=off  XmcBlockStatus=1  maskContainerNames=tabcontainer1  block_type=addsub  block_config=sysgen:Addsub_config
  Out2_r : Outport
  Out2_i : Outport  Port=2
  Out1_r : Outport  Port=3
  Out1_i : Outport  Port=4
  wires:
  AddSub2/1 -> Out2_r/1
  AddSub1/1 -> Out2_i/1
  AddSub3/1 -> Out1_r/1
  AddSub4/1 -> Out1_i/1
  ur/1 -> AddSub2/1, AddSub3/1
  ui/1 -> AddSub1/1, AddSub4/1
  vr/1 -> AddSub2/2, AddSub3/2
  vi/1 -> AddSub1/2, AddSub4/2

== system sys1/SAR/stream/stream_ifft/stage3/Multiplexer ==
  r2 : Inport
  i2 : Inport  Port=2
  r1 : Inport  Port=3
  i1 : Inport  Port=4
  cnt : Inport  Port=5
  BitBasher : hdlBasic/BitBasher  bitexpr=a={b[12]}  display_expr=on  sr_1=a  arith_type1=Unsigned  bin_pt1=0  sr_2=2  arith_type2=Unsigned  bin_pt2=0  sr_3=3  arith_type3=Unsigned  bin_pt3=0  sr_4=4  arith_type4=Unsigned  bin_pt4=0  XmcBlockStatus=1  maskContainerNames=group1  block_type=bitbasher  block_config=sysgen:BitBasher_config
  Delay1 : hdlBasic/Delay  rst=off  en=off  latency=7  reg_retiming=off  XmcBlockStatus=1  maskContainerNames=group1  block_type=delay  block_config=sysgen:Delay_config
  Inverter : hdlBasic/Inverter  en=off  latency=0  XmcBlockStatus=1  maskContainerNames=group2  block_type=inv  block_config=sysgen:Inverter_config
  Mux : hdlBasic/Mux  inputs=2  en=off  latency=0  precision=Full  arith_type=Unsigned  n_bits=16  bin_pt=14  quantization=Truncate  overflow=Wrap  XmcBlockStatus=1  maskContainerNames=tabcontainer1  block_type=mux  block_config=sysgen:Mux_config
  Mux1 : hdlBasic/Mux  inputs=2  en=off  latency=0  precision=Full  arith_type=Unsigned  n_bits=16  bin_pt=14  quantization=Truncate  overflow=Wrap  XmcBlockStatus=1  maskContainerNames=tabcontainer1  block_type=mux  block_config=sysgen:Mux_config
  rr : Outport
  ii : Outport  Port=2
  wires:
  Delay1/1 -> Mux1/1, Mux/1
  Inverter/1 -> Delay1/1
  r1/1 -> Mux/2
  r2/1 -> Mux/3
  i2/1 -> Mux1/3
  i1/1 -> Mux1/2
  cnt/1 -> BitBasher/1
  Mux/1 -> rr/1
  Mux1/1 -> ii/1
  BitBasher/1 -> Inverter/1

== system sys1/SAR/stream/stream_ifft/stage3/Twiddle1 ==
  r : Inport
  i : Inport  Port=2
  cnt : Inport  Port=3
  BitBasher1 : hdlBasic/BitBasher  bitexpr=a={b[11:10]}  display_expr=on  sr_1=a  arith_type1=Unsigned  bin_pt1=0  sr_2=2  arith_type2=Unsigned  bin_pt2=0  sr_3=3  arith_type3=Unsigned  bin_pt3=0  sr_4=4  arith_type4=Unsigned  bin_pt4=0  XmcBlockStatus=1  maskContainerNames=group1  block_type=bitbasher  block_config=sysgen:BitBasher_config
  Complex Multiplier 6.0 : hdlDSPIP/Complex Multiplier 6.0   hasatlast=off  hasatuser=off  atuserwidth=1  hasbtlast=off  hasbtuser=off  btuserwidth=1  multtype=Use_Mults  optimizegoal=Resources  flowcontrol=NonBlocking  outputwidth=32  roundmode=Truncate  hasctrltlast=off  hasctrltuser=off  ctrltuserwidth=1  outtlastbehv=Null  latencyconfig=Manual  minimumlatency=6  aclken=off  aresetn=off  trim_axipin_name=on  simulation_type=hybrid_sim  simulation_model=sysgen:cmpy_v6_0  data_path_portlist={ 's_axis_a_tdata_real', 's_axis_a_tdata_imag', 's_axis_b_tdata_real', 's_axis_b_tdata_imag', 's_axis_ctrl_tdata_rounding_bit', 'm_axis_dout_tdata_real', 'm_axis_dout_tdata_imag' }  aportwidth=63  bportwidth=63  ip_name=Complex Multiplier  ip_version=6.0  dsptool_ready=true  ipcore_usecache=true  ipcore_useipmodelcache=true  ipcore_verbose=false  ipcore_latency_parameter='minimumlatency'  wrapper_available=true  port_translation_map={ 'aclken' => 'en', 'aresetn' => 'rst'}  XmcBlockStatus=1  maskContainerNames=tabcontainer1  block_type=cmpy_v6_0  block_config=sysgen:rodinimport_config
  Constant2 : hdlBasic/Constant  const=1  gui_display_data_type=Boolean  arith_type=Boolean  n_bits=16  bin_pt=14  preci_type=Single  exp_width=8  frac_width=24  explicit_period=on  period=ts  XmcBlockStatus=1  maskContainerNames=tabcontainer1  block_type=constant  block_config=sysgen:Constant_config
  Constant3 : hdlBasic/Constant  const=1  gui_display_data_type=Boolean  arith_type=Boolean  n_bits=16  bin_pt=14  preci_type=Single  exp_width=8  frac_width=24  explicit_period=on  period=ts  XmcBlockStatus=1  maskContainerNames=tabcontainer1  block_type=constant  block_config=sysgen:Constant_config
  Convert : hdlBasic/Convert  gui_display_data_type=Fixed-point  arith_type=Signed (2's comp)  n_bits=16  bin_pt=0  float_type=Single  exp_bits=8  fraction_bits=24  quantization="Round  (unbiased: +/- Inf)"  overflow=Flag as error  en=off  latency=0  pipeline=off  XmcBlockStatus=1  maskContainerNames=group2  block_type=convert  block_config=sysgen:Convert_config  block_width=595  block_height=885
  Convert1 : hdlBasic/Convert  gui_display_data_type=Fixed-point  arith_type=Signed (2's comp)  n_bits=16  bin_pt=0  float_type=Single  exp_bits=8  fraction_bits=24  quantization="Round  (unbiased: +/- Inf)"  overflow=Flag as error  en=off  latency=0  pipeline=off  XmcBlockStatus=1  maskContainerNames=group2  block_type=convert  block_config=sysgen:Convert_config  block_width=595  block_height=885
  ROM : hdlBasic/ROM  depth=length(ww3)  initVector=real(ww3)  distributed_mem=Block RAM  rst=off  init_reg=0  en=off  latency=1  gui_display_data_type=Fixed-point  arith_type="Signed  (2's comp)"  n_bits=17  bin_pt=15  preci_type=Single  exp_width=8  frac_width=24  optimize=Area  use_rpm=on  simulation_type=fast_sim  XmcBlockStatus=1  maskContainerNames=tabcontainer1  block_type=sprom  block_config=sysgen:SPROM_config
  ROM1 : hdlBasic/ROM  depth=length(ww3)  initVector=imag(ww3)  distributed_mem=Block RAM  rst=off  init_reg=0  en=off  latency=1  gui_display_data_type=Fixed-point  arith_type="Signed  (2's comp)"  n_bits=17  bin_pt=15  preci_type=Single  exp_width=8  frac_width=24  optimize=Area  use_rpm=on  simulation_type=fast_sim  XmcBlockStatus=1  maskContainerNames=tabcontainer1  block_type=sprom  block_config=sysgen:SPROM_config
  rr : Outport
  ii : Outport  Port=2
  wires:
  ROM/1 -> Complex Multiplier 6.0/6
  ROM1/1 -> Complex Multiplier 6.0/5
  cnt/1 -> BitBasher1/1
  r/1 -> Complex Multiplier 6.0/3
  i/1 -> Complex Multiplier 6.0/2
  Convert/1 -> ii/1
  Convert1/1 -> rr/1
  Complex Multiplier 6.0/2 -> Convert/1
  Complex Multiplier 6.0/3 -> Convert1/1
  BitBasher1/1 -> ROM1/1, ROM/1
  Constant3/1 -> Complex Multiplier 6.0/4
  Constant2/1 -> Complex Multiplier 6.0/1

== system sys1/SAR/stream/stream_ifft/stage3/delay ==
  r : Inport
  i : Inport  Port=2
  cnt : Inport  Port=3
  r1 : Inport  Port=4
  i1 : Inport  Port=5
  BitBasher : hdlBasic/BitBasher  bitexpr=a={b[12]}  display_expr=off  sr_1=a  arith_type1=Unsigned  bin_pt1=0  sr_2=2  arith_type2=Unsigned  bin_pt2=0  sr_3=3  arith_type3=Unsigned  bin_pt3=0  sr_4=4  arith_type4=Unsigned  bin_pt4=0  XmcBlockStatus=1  maskContainerNames=group1  block_type=bitbasher  block_config=sysgen:BitBasher_config
  Delay4 : hdlBasic/Delay  rst=off  en=off  latency=6  reg_retiming=off  XmcBlockStatus=1  maskContainerNames=group1  block_type=delay  block_config=sysgen:Delay_config
  Delay6 : hdlBasic/Delay  rst=off  en=off  latency=6  reg_retiming=off  XmcBlockStatus=1  maskContainerNames=group1  block_type=delay  block_config=sysgen:Delay_config
  Delay9 : hdlBasic/Delay  rst=off  en=off  latency=7  reg_retiming=off  XmcBlockStatus=1  maskContainerNames=group1  block_type=delay  block_config=sysgen:Delay_config
  Inverter : hdlBasic/Inverter  en=off  latency=0  XmcBlockStatus=1  maskContainerNames=group2  block_type=inv  block_config=sysgen:Inverter_config
  Mux : hdlBasic/Mux  inputs=2  en=off  latency=0  precision=Full  arith_type=Unsigned  n_bits=16  bin_pt=14  quantization=Truncate  overflow=Wrap  XmcBlockStatus=1  maskContainerNames=tabcontainer1  block_type=mux  block_config=sysgen:Mux_config
  Mux1 : hdlBasic/Mux  inputs=2  en=off  latency=0  precision=Full  arith_type=Unsigned  n_bits=16  bin_pt=14  quantization=Truncate  overflow=Wrap  XmcBlockStatus=1  maskContainerNames=tabcontainer1  block_type=mux  block_config=sysgen:Mux_config
  delay : Subsystem
  delay1 : Subsystem
  rr : Outport
  ii : Outport  Port=2
  wires:
  Delay6/1 -> Mux1/3
  Delay4/1 -> Mux/3
  Delay9/1 -> Mux1/1, Mux/1
  r1/1 -> Mux/2
  i/1 -> Delay6/1
  Mux1/1 -> delay1/1(in)
  BitBasher/1 -> Inverter/1
  i1/1 -> Mux1/2
  r/1 -> Delay4/1
  delay/1(out) -> rr/1
  delay1/1(out) -> ii/1
  Mux/1 -> delay/1(in)
  cnt/1 -> BitBasher/1
  Inverter/1 -> Delay9/1

== system sys1/SAR/stream/stream_ifft/stage4/BF ==
  ur : Inport
  ui : Inport  Port=2
  vr : Inport  Port=3
  vi : Inport  Port=4
  AddSub1 : hdlBasic/AddSub  mode=Addition  use_carryin=off  use_carryout=off  en=off  latency=0  precision=User Defined  arith_type="Signed  (2's comp)"  n_bits=16  bin_pt=0  quantization="Round  (unbiased: +/- Inf)"  overflow=Flag as error  use_behavioral_HDL=off  hw_selection=Fabric  pipelined=off  XmcBlockStatus=1  maskContainerNames=tabcontainer1  block_type=addsub  block_config=sysgen:Addsub_config
  AddSub2 : hdlBasic/AddSub  mode=Addition  use_carryin=off  use_carryout=off  en=off  latency=0  precision=User Defined  arith_type="Signed  (2's comp)"  n_bits=16  bin_pt=0  quantization="Round  (unbiased: +/- Inf)"  overflow=Flag as error  use_behavioral_HDL=off  hw_selection=Fabric  pipelined=off  XmcBlockStatus=1  maskContainerNames=tabcontainer1  block_type=addsub  block_config=sysgen:Addsub_config
  AddSub3 : hdlBasic/AddSub  mode=Subtraction  use_carryin=off  use_carryout=off  en=off  latency=0  precision=User Defined  arith_type="Signed  (2's comp)"  n_bits=16  bin_pt=0  quantization="Round  (unbiased: +/- Inf)"  overflow=Flag as error  use_behavioral_HDL=off  hw_selection=Fabric  pipelined=off  XmcBlockStatus=1  maskContainerNames=tabcontainer1  block_type=addsub  block_config=sysgen:Addsub_config
  AddSub4 : hdlBasic/AddSub  mode=Subtraction  use_carryin=off  use_carryout=off  en=off  latency=0  precision=User Defined  arith_type="Signed  (2's comp)"  n_bits=16  bin_pt=0  quantization="Round  (unbiased: +/- Inf)"  overflow=Flag as error  use_behavioral_HDL=off  hw_selection=Fabric  pipelined=off  XmcBlockStatus=1  maskContainerNames=tabcontainer1  block_type=addsub  block_config=sysgen:Addsub_config
  Out2_r : Outport
  Out2_i : Outport  Port=2
  Out1_r : Outport  Port=3
  Out1_i : Outport  Port=4
  wires:
  AddSub2/1 -> Out2_r/1
  AddSub1/1 -> Out2_i/1
  AddSub3/1 -> Out1_r/1
  AddSub4/1 -> Out1_i/1
  ur/1 -> AddSub2/1, AddSub3/1
  ui/1 -> AddSub1/1, AddSub4/1
  vr/1 -> AddSub2/2, AddSub3/2
  vi/1 -> AddSub1/2, AddSub4/2
